simulink model "Three_phase_fully_controlled_converter_fed DC_motor"  (R2024a)
settings: Solver=VariableStepAuto  StartTime=0.0  StopTime=0.6  RelTol=1e-3
libraries: spsThyristorLib x6, spsDCMachineLib x1, spsDCVoltageSourceLib x1, spsGroundLib x1, spsThreePhaseProgrammableVoltageSourceLib x1, spsVoltageMeasurementLib x1, sps_lib x1
settings Model: Creator=haris  LastModifiedBy=haris

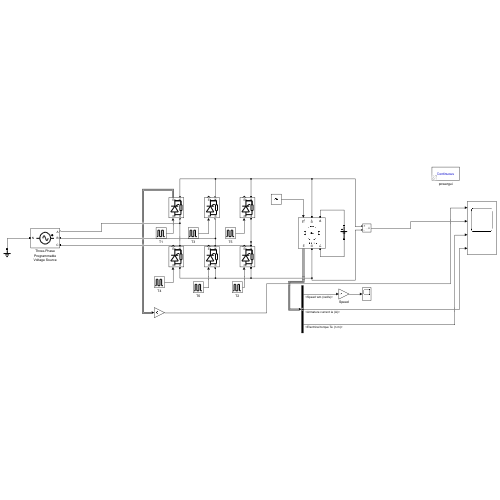
[thumbnail: Simulink's stored preview of the top-level diagram]
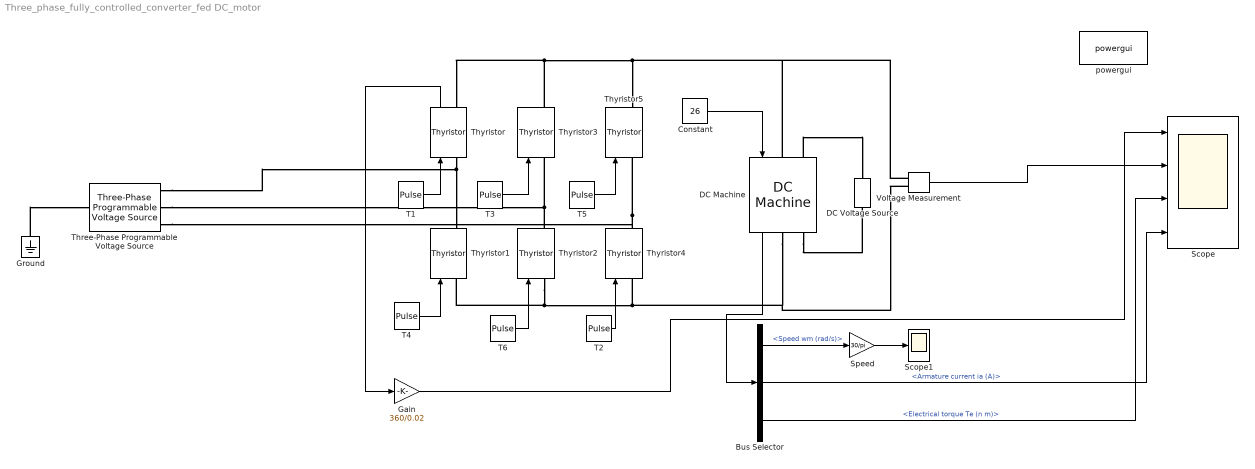
== system Three_phase_fully_controlled_converter_fed DC_motor ==
  Bus Selector : BusSelector  OutputSignals=Speed wm (rad/s),Armature current ia (A),Electrical torque Te (n m)
  Constant : Constant  Value=26
  DC Machine : spsDCMachineLib/DC Machine  PresetModel=01: 5HP 240V 1750RPM Field:300V  MechanicalLoad=Torque TL  FieldType=Wound  ShowDetailedParameters=on  MeasurementBus=off  RLa=[2.581 0.028]  RLf=[281.2 156]  Laf=0.9483  MachineConstant=Torque constant (N.m/A)  Ke=1.8  Kt=1.8  J=0.02215  Bm=0.002953  Tf=0.5161  w0=0  Ifinit=1.06685632871799  TsPowergui=0  TsBlock=-1
  DC Voltage Source : spsDCVoltageSourceLib/DC Voltage Source  Amplitude=300  Measurements=None
  Gain : Gain  Gain=360/0.02
  Ground : spsGroundLib/Ground  LConnTagsString=a
  Scope : Scope  NumInputPorts=4
  Scope1 : Scope
  Speed : Gain  Gain=30/pi
  T1 : DiscretePulseGenerator  PulseType=Time based  Period=0.02  PulseWidth=50  PhaseDelay=0.02*(0/360)
  T2 : DiscretePulseGenerator  PulseType=Time based  Period=0.02  PulseWidth=50  PhaseDelay=0.02*(60/360)
  T3 : DiscretePulseGenerator  PulseType=Time based  Period=0.02  PulseWidth=50  PhaseDelay=0.02*(120/360)
  T4 : DiscretePulseGenerator  PulseType=Time based  Period=0.02  PulseWidth=50  PhaseDelay=0.02*(180/360)
  T5 : DiscretePulseGenerator  PulseType=Time based  Period=0.02  PulseWidth=50  PhaseDelay=0.02*(240/360)
  T6 : DiscretePulseGenerator  PulseType=Time based  Period=0.02  PulseWidth=50  PhaseDelay=0.02*(300/360)
  Three-Phase Programmable Voltage Source : spsThreePhaseProgrammableVoltageSourceLib/Three-Phase Programmable Voltage Source  PositiveSequence="[188  0 50]"  VariationEntity=None  VariationType=Table of time-amplitude pairs  VariationTypeAlt=Step  VariationStep=0.5  VariationRate=10  VariationMagnitude=0.3  VariationFrequency=2  VariationTiming=[1 2]  VariationPhaseA=off  Amplitudes=[1 0.8 1.2 1.0]  TimeValues=[0 0.1 0.15 0.2]  HarmonicGeneration=off  HarmonicA=[3 0.2 -25 0]  HarmonicB=[2 0.15 35 2]  Timing="[0.05  3]"  BusType=swing  Pref=0  Qref=0  Qmin=-inf  Qmax=inf
  Thyristor{,1..5} (6 alike) : spsThyristorLib/Thyristor  Ron=0.001  Lon=0  Vf=0.8  IC=0  Rs=500  Cs=250e-9  Measurements=on
  Voltage Measurement : spsVoltageMeasurementLib/Voltage Measurement  PhasorSimulation=off  OutputType=Complex  PSBequivalent=0
  powergui : sps_lib/powergui  Priority=1  SimulationMode=Continuous  SampleTime=50e-6  frequency=60  Iterations=50  frequencyindice=50  Pbase=100e6  ErrMax=1e-4  UnitsV=kV  UnitsW=MW  buscounter=0  FunctionMessages=off  echomessages=off  EnableUseOfTLC=off  CurrentSourceSwitches=off  DisableSnubberDevices=off  DisableRonSwitches=off  DisableVfSwitches=off  DisplayEquations=off  AutomaticDiscreteSolvers=off  SolverType=Tustin/Backward Euler (TBE)  Interpol=off  ExternalGateDelay=off  methode=off  Ts=100  x0status=blocks  SPID=on  SwTol=0  HookPort=off  NonlinearTolerance=1e-4  nMaxIteration=100  ContinueOnMaxIteration=off  RestoreLinks=warning  ResistiveCurrentMeasurement=off  Frange=[0:2:500]  Ylog=off  Xlog=on  ShowGrid=off  save=off  variable=ZData  structure=0  ZoomFFT=off  StartTime=0.0  cycles=1  DisplayStyle=1  fundamental=60  FreqAxis=off  MaxFrequency=1000  frequencyindicesteady=1  RmsSteady=1  display=off
  wires:
  DC Machine/1 -> Bus Selector/1
  Voltage Measurement/1 -> Scope/2
  Bus Selector/2 -> Scope/4  "<Armature current ia (A)>"
  Constant/1 -> DC Machine/1
  T1/1 -> Thyristor/1
  T3/1 -> Thyristor3/1
  T5/1 -> Thyristor5/1
  T4/1 -> Thyristor1/1
  T6/1 -> Thyristor2/1
  T2/1 -> Thyristor4/1
  Thyristor/1 -> Gain/1
  Gain/1 -> Scope/1
  Bus Selector/3 -> Scope/3  "<Electrical torque Te (n m)>"
  Bus Selector/1 -> Speed/1  "<Speed wm (rad/s)>"
  Speed/1 -> Scope1/1
  connections:
  Ground/LConn1 -- Three-Phase Programmable Voltage Source/LConn1
  Thyristor2/RConn1 -- Thyristor3/LConn1 -- Three-Phase Programmable Voltage Source/RConn2
  Thyristor4/RConn1 -- Three-Phase Programmable Voltage Source/RConn3 -- Thyristor5/LConn1
  Thyristor/LConn1 -- Three-Phase Programmable Voltage Source/RConn1 -- Thyristor1/RConn1
  Thyristor2/LConn1 -- DC Machine/RConn1 -- Voltage Measurement/LConn2 -- Thyristor4/LConn1 -- Thyristor1/LConn1
  Thyristor3/RConn1 -- DC Machine/LConn1 -- Voltage Measurement/LConn1 -- Thyristor5/RConn1 -- Thyristor/RConn1
  DC Machine/LConn2 -- DC Voltage Source/RConn1
  DC Machine/RConn2 -- DC Voltage Source/LConn1
